simulink model "QD2_DroneStack_PID_2021a"  (R2022a)
settings: Solver=ode1  StartTime=0.0  StopTime=inf  FixedStep=1/1000  RelTol=1e-3  EnableMultiTasking=on
InitFcn:
  | Motor_Mapping_7_Inch
model workspace (MAT data in the model file):
  target_system = 1
values from neighbouring files (symbols this model uses):
  KT = [0.03616,0.117,-0.01215]    [Motor_Mapping_7_Inch.m]
  Motor_Matrix = [ 0.25   -1/(2*L_Roll)    1/(2*L_Pitch)    K_Tau/4;                  0.25   -1/(2*L_Roll)   -1/(2*L_Pitch)   -K_Tau/4;                  0.25    1/(2*L_Roll)    1/(2*L_Pitch)   -K_Tau/4;                  0.25    1/(2*L_Roll)   -1/(2*L_Pitch)    K_Tau/4]    [Motor_Mapping_7_Inch.m]
undefined symbols (not defined in the file or in its folder): _Commander, _QDrone2, _Stabilizer, datetime, HIL, lf, log_, m, n, qc_get_step_size, s, saved_data
libraries: quarc_library x94, simulink x27, simulink_extras x9
(part 3 of 4)

== system QD2_DroneStack_PID_2021a/COMMANDER (ANGLE MODE)/STATE MACHINE SIGNALS/Generate Extra Messages for Console ==
  time (s) : Inport
  Signal Triggers : Inport  Port=2
  Boolean Edge-Based Triggered Print : Subsystem  TreatAsAtomicUnit=on
  Matrix Concatenate : Concatenate  NumInputs=3  Mode=Multidimensional array  ConcatenateDimension=2
  String Constant12 : quarc_library/Strings/String Constant  string_value=DRONE DISARMED  evaluate_string=off  string_type=text  max_length=80  sample_time=inf  variable_size=off
      settings: AttributesFormatString="\"DRONE DISARMED\""  SourceProductName=QUARC Targets
  String Constant13 : quarc_library/Strings/String Constant  string_value=DRONE LANDING  evaluate_string=off  string_type=text  max_length=80  sample_time=inf  variable_size=off
      settings: AttributesFormatString="\"DRONE LANDING\""  SourceProductName=QUARC Targets
  String Constant16 : quarc_library/Strings/String Constant  string_value=INITIALIZATION FINISHED  evaluate_string=off  string_type=text  max_length=80  sample_time=inf  variable_size=off
      settings: AttributesFormatString="\"INITIALIZATION FINISHED\""  SourceProductName=QUARC Targets
  Terminator : Terminator
  wires:
  Boolean Edge-Based Triggered Print/1(Out1) -> Terminator/1
  String Constant13/1 -> Matrix Concatenate/3
  String Constant12/1 -> Matrix Concatenate/2
  String Constant16/1 -> Matrix Concatenate/1
  Signal Triggers/1 -> Boolean Edge-Based Triggered Print/1(Signal Enable)
  time (s)/1 -> Boolean Edge-Based Triggered Print/3(time (s))
  Matrix Concatenate/1 -> Boolean Edge-Based Triggered Print/2(Message)

== system QD2_DroneStack_PID_2021a/COMMANDER (ANGLE MODE)/STATE MACHINE SIGNALS/Generate State Messages for Console ==
  time (s) : Inport
  DroneState [1-9] : Inport  Port=2
  Detect Change : simulink/Logic and Bit Operations/Detect Change  vinit=0  OutDataTypeStr=boolean
  Multiport Switch : MultiPortSwitch  Inputs=9  SaturateOnIntegerOverflow=off  InputSameDT=off
  String Constant1 : quarc_library/Strings/String Constant  string_value=DRONE ARMED  evaluate_string=off  string_type=text  max_length=80  sample_time=inf  variable_size=off
      settings: AttributesFormatString="\"DRONE ARMED\""  SourceProductName=QUARC Targets
  String Constant2 : quarc_library/Strings/String Constant  string_value=DRONE TAKEOFF THROTTLE  evaluate_string=off  string_type=text  max_length=80  sample_time=inf  variable_size=off
      settings: AttributesFormatString="\"DRONE TAKEOFF THROTTLE\""  SourceProductName=QUARC Targets
  String Constant3 : quarc_library/Strings/String Constant  string_value=DRONE TAKEOFF HEIGHT STATE  evaluate_string=off  string_type=text  max_length=80  sample_time=inf  variable_size=off
      settings: AttributesFormatString="\"DRONE TAKEOFF HEIGHT STATE\""  SourceProductName=QUARC Targets
  String Constant4 : quarc_library/Strings/String Constant  string_value=ERROR - DRONE EMERGENCY STOP  evaluate_string=off  string_type=text  max_length=80  sample_time=inf  variable_size=off
      settings: AttributesFormatString="\"ERROR - DRONE EMERGENCY STOP\""  SourceProductName=QUARC Targets
  String Constant5 : quarc_library/Strings/String Constant  string_value=DRONE IDLE - WAITING TO BE ARMED  evaluate_string=off  string_type=text  max_length=80  sample_time=inf  variable_size=off
      settings: AttributesFormatString="\"DRONE IDLE - WAITING TO BE ARMED\""  SourceProductName=QUARC Targets
  String Constant6 : quarc_library/Strings/String Constant  string_value=DRONE IS IN FLIGHT STATE  evaluate_string=off  string_type=text  max_length=80  sample_time=inf  variable_size=off
      settings: AttributesFormatString="\"DRONE IS IN FLIGHT STATE\""  SourceProductName=QUARC Targets
  String Constant7 : quarc_library/Strings/String Constant  string_value=EMERGENCY STOP WAS PRESSED ON JOYSTICK  evaluate_string=off  string_type=text  max_length=80  sample_time=inf  variable_size=off
      settings: AttributesFormatString="\"EMERGENCY STOP WAS PRESSED ON JOYSTICK\""  SourceProductName=QUARC Targets
  String Constant8 : quarc_library/Strings/String Constant  string_value=FLIGHT FINISHED DRONE IS DISABLED  evaluate_string=off  string_type=text  max_length=80  sample_time=inf  variable_size=off
      settings: AttributesFormatString="\"FLIGHT FINISHED DRONE IS DISABLED\""  SourceProductName=QUARC Targets
  String Constant9 : quarc_library/Strings/String Constant  string_value=DRONE IS AUTO LANDING  evaluate_string=off  string_type=text  max_length=80  sample_time=inf  variable_size=off
      settings: AttributesFormatString="\"DRONE IS AUTO LANDING\""  SourceProductName=QUARC Targets
  Triggered Subsystem : Subsystem  TreatAsAtomicUnit=on
  wires:
  Detect Change/1 -> Triggered Subsystem/Trigger
  String Constant5/1 -> Multiport Switch/2
  String Constant8/1 -> Multiport Switch/10
  String Constant7/1 -> Multiport Switch/9
  String Constant4/1 -> Multiport Switch/8
  String Constant9/1 -> Multiport Switch/7
  String Constant6/1 -> Multiport Switch/6
  String Constant3/1 -> Multiport Switch/5
  String Constant2/1 -> Multiport Switch/4
  String Constant1/1 -> Multiport Switch/3
  time (s)/1 -> Triggered Subsystem/2(Time (s))
  Multiport Switch/1 -> Triggered Subsystem/3(Message)
  DroneState [1-9]/1 -> Detect Change/1, Triggered Subsystem/1(Value), Multiport Switch/1

== system QD2_DroneStack_PID_2021a/COMMANDER (ANGLE MODE)/STATE MACHINE SIGNALS/Generate Warning Messages for Console ==
  time (s) : Inport
  errors [8] : Inport  Port=2
  Boolean Value-Based Triggered Print : Subsystem  TreatAsAtomicUnit=on
  Matrix Concatenate : Concatenate  NumInputs=9  Mode=Multidimensional array  ConcatenateDimension=2
  String Constant : quarc_library/Strings/String Constant  string_value=Commander: Low Battery  evaluate_string=off  string_type=text  max_length=80  sample_time=inf  variable_size=off
      settings: AttributesFormatString="\"Commander: Low Battery\""  SourceProductName=QUARC Targets
  String Constant1 : quarc_library/Strings/String Constant  string_value=Commander: Sensor Failure  evaluate_string=off  string_type=text  max_length=80  sample_time=inf  variable_size=off
      settings: AttributesFormatString="\"Commander: Sensor Failure\""  SourceProductName=QUARC Targets
  String Constant2 : quarc_library/Strings/String Constant  string_value=Commander: Host Stream Issue / Problem with communication  evaluate_string=off  string_type=text  max_length=80  sample_time=inf  variable_size=off
      settings: AttributesFormatString="\"Commander: Host Stream Issue / Problem with communication\""  SourceProductName=QUARC Targets
  String Constant3 : quarc_library/Strings/String Constant  string_value=Commander: Joystick Issue  evaluate_string=off  string_type=text  max_length=80  sample_time=inf  variable_size=off
      settings: AttributesFormatString="\"Commander: Joystick Issue\""  SourceProductName=QUARC Targets
  String Constant4 : quarc_library/Strings/String Constant  string_value=Commander: Optitrack isn't tracking  evaluate_string=off  string_type=text  max_length=80  sample_time=inf  variable_size=off
      settings: AttributesFormatString="\"Commander: Optitrack isn't tracking\""  SourceProductName=QUARC Targets
  String Constant5 : quarc_library/Strings/String Constant  string_value=Commander: Flying low  evaluate_string=off  string_type=text  max_length=80  sample_time=inf  variable_size=off
      settings: AttributesFormatString="\"Commander: Flying low\""  SourceProductName=QUARC Targets
  String Constant6 : quarc_library/Strings/String Constant  string_value=Commander: Flying high  evaluate_string=off  string_type=text  max_length=80  sample_time=inf  variable_size=off
      settings: AttributesFormatString="\"Commander: Flying high\""  SourceProductName=QUARC Targets
  String Constant7 : quarc_library/Strings/String Constant  string_value=Commander: Emergency Stop Triggered  evaluate_string=off  string_type=text  max_length=80  sample_time=inf  variable_size=off
      settings: AttributesFormatString="\"Commander: Emergency Stop Triggered\""  SourceProductName=QUARC Targets
  String Constant8 : quarc_library/Strings/String Constant  string_value=Commander: Takeoff triggered before armed drone  evaluate_string=off  string_type=text  max_length=80  sample_time=inf  variable_size=off
      settings: AttributesFormatString="\"Commander: Takeoff triggered before armed drone\""  SourceProductName=QUARC Targets
  Terminator : Terminator
  wires:
  time (s)/1 -> Boolean Value-Based Triggered Print/3(time (s))
  errors [8]/1 -> Boolean Value-Based Triggered Print/1(Signal Enable)
  Matrix Concatenate/1 -> Boolean Value-Based Triggered Print/2(Message)
  String Constant/1 -> Matrix Concatenate/1
  String Constant1/1 -> Matrix Concatenate/2
  String Constant2/1 -> Matrix Concatenate/3
  String Constant3/1 -> Matrix Concatenate/4
  Boolean Value-Based Triggered Print/1(Out1) -> Terminator/1
  String Constant7/1 -> Matrix Concatenate/9
  String Constant6/1 -> Matrix Concatenate/8
  String Constant5/1 -> Matrix Concatenate/7
  String Constant4/1 -> Matrix Concatenate/6
  String Constant8/1 -> Matrix Concatenate/5

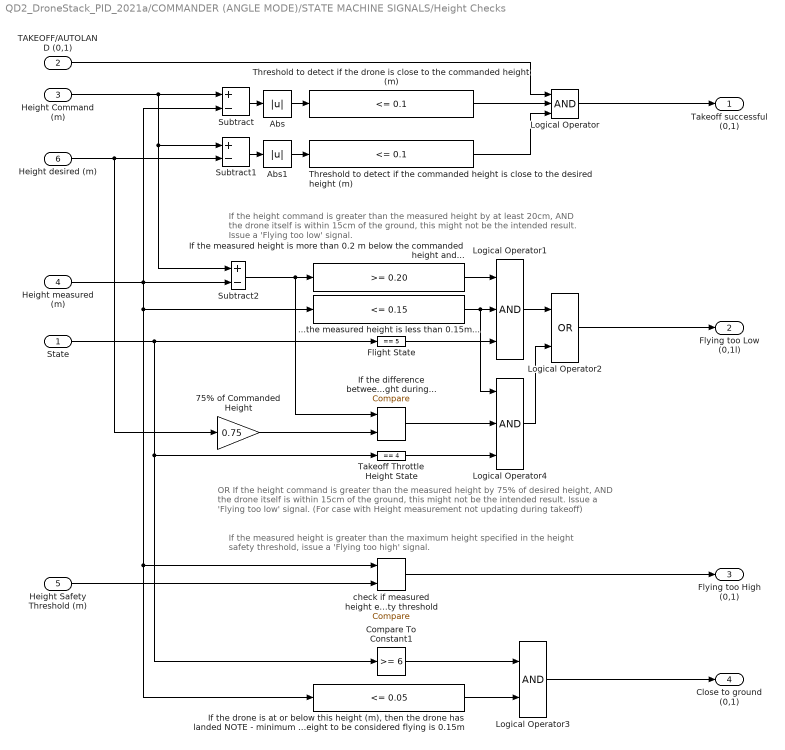
== system QD2_DroneStack_PID_2021a/COMMANDER (ANGLE MODE)/STATE MACHINE SIGNALS/Height Checks ==
  note: If the height command is greater than the measured height by at least 20cm, AND the drone itself is
      | within 15cm of the ground, this might not be the intended result. Issue a 'Flying too low' signal.
  note: If the measured height is greater than the maximum height specified in the height safety threshold,
      | issue a 'Flying too high' signal.
  note: OR If the height command is greater than the measured height by 75% of desired height, AND
      | the drone itself is within 15cm of the ground, this might not be the intended result. Issue a 'Flying too low' signal.
      | (For case with Height measurement not updating during takeoff)
  State : Inport
  TAKEOFF/AUTOLAND (0,1) : Inport  Port=2
  Height Command (m) : Inport  Port=3
  Height measured (m) : Inport  Port=4
  Height Safety Threshold (m) : Inport  Port=5
  Height desired (m) : Inport  Port=6
  ...the measured height is less than 0.15m... : simulink/Logic and Bit Operations/Compare To Constant  relop=<=  const=0.15  OutDataTypeStr=boolean
  75% of Commanded Height : Gain  Gain=0.75
  Abs : Abs  SaturateOnIntegerOverflow=off
  Abs1 : Abs  SaturateOnIntegerOverflow=off
  Compare To Constant1 : simulink/Logic and Bit Operations/Compare To Constant  relop=>=  const=6  OutDataTypeStr=boolean
  Flight State : simulink/Logic and Bit Operations/Compare To Constant  relop===  const=5  OutDataTypeStr=boolean
  If the difference between the measured and commanded height is greater than 75% of the commanded height during... : quarc_library/Logic Operations/Compare  operator=>=  output_data_type=boolean
      settings: SourceProductName=QUARC Targets
  "If the drone is at or below this height (m), then the drone has landed NOTE - minimum height to be considered flying is 0.15m   " : simulink/Logic and Bit Operations/Compare To Constant  relop=<=  const=0.05  OutDataTypeStr=boolean
  If the measured height is more than 0.2 m below the commanded height and... : simulink/Logic and Bit Operations/Compare To Constant  relop=>=  const=0.20  OutDataTypeStr=boolean
  Logical Operator : Logic  Inputs=3  AllPortsSameDT=off  OutDataTypeStr=boolean
  Logical Operator1 : Logic  Inputs=3  AllPortsSameDT=off  OutDataTypeStr=boolean
  Logical Operator2 : Logic  Operator=OR  AllPortsSameDT=off  OutDataTypeStr=boolean
  Logical Operator3 : Logic  AllPortsSameDT=off  OutDataTypeStr=boolean
  Logical Operator4 : Logic  Inputs=3  AllPortsSameDT=off  OutDataTypeStr=boolean
  Subtract : Sum  Inputs=+-
  Subtract1 : Sum  Inputs=+-
  Subtract2 : Sum  Inputs=+-
  Takeoff Throttle Height State : simulink/Logic and Bit Operations/Compare To Constant  relop===  const=4  OutDataTypeStr=boolean
  Threshold to detect if the commanded height is close to the desired height (m) : simulink/Logic and Bit Operations/Compare To Constant  relop=<=  const=0.1  OutDataTypeStr=boolean
  Threshold to detect if the drone is close to the commanded height (m) : simulink/Logic and Bit Operations/Compare To Constant  relop=<=  const=0.1  OutDataTypeStr=boolean
  check if measured height exceeds maximum height safety threshold : quarc_library/Logic Operations/Compare  operator=>=  output_data_type=boolean
      settings: SourceProductName=QUARC Targets
  Takeoff successful (0,1) : Outport  VectorParamsAs1DForOutWhenUnconnected=off
  Flying too Low (0,1l) : Outport  Port=2  VectorParamsAs1DForOutWhenUnconnected=off
  Flying too High (0,1) : Outport  Port=3  VectorParamsAs1DForOutWhenUnconnected=off
  Close to ground (0,1) : Outport  Port=4  VectorParamsAs1DForOutWhenUnconnected=off
  wires:
  Logical Operator/1 -> Takeoff successful (0,1)/1
  Logical Operator2/1 -> Flying too Low (0,1l)/1
  Subtract1/1 -> Abs1/1
  Threshold to detect if the commanded height is close to the desired height (m)/1 -> Logical Operator/3
  Abs/1 -> Threshold to detect if the drone is close to the commanded height (m)/1
  Threshold to detect if the drone is close to the commanded height (m)/1 -> Logical Operator/2
  Abs1/1 -> Threshold to detect if the commanded height is close to the desired height (m)/1
  Height desired (m)/1 -> 75% of Commanded Height/1, Subtract1/2
  TAKEOFF/AUTOLAND (0,1)/1 -> Logical Operator/1
  Subtract/1 -> Abs/1
  If the measured height is more than 0.2 m below the commanded height and.../1 -> Logical Operator1/1
  Logical Operator1/1 -> Logical Operator2/1
  Height Command (m)/1 -> Subtract1/1, Subtract2/1, Subtract/1
  ...the measured height is less than 0.15m.../1 -> Logical Operator4/1, Logical Operator1/2
  check if measured height exceeds maximum height safety threshold/1 -> Flying too High (0,1)/1
  Height Safety Threshold (m)/1 -> check if measured height exceeds maximum height safety threshold/2
  State/1 -> Flight State/1, Takeoff Throttle Height State/1, Compare To Constant1/1
  Logical Operator3/1 -> Close to ground (0,1)/1
  "If the drone is at or below this height (m), then the drone has landed NOTE - minimum height to be considered flying is 0.15m   "/1 -> Logical Operator3/2
  Compare To Constant1/1 -> Logical Operator3/1
  Height measured (m)/1 -> Subtract/2, ...the measured height is less than 0.15m.../1, "If the drone is at or below this height (m), then the drone has landed NOTE - minimum height to be considered flying is 0.15m   "/1, check if measured height exceeds maximum height safety threshold/1, Subtract2/2
  Logical Operator4/1 -> Logical Operator2/2
  Flight State/1 -> Logical Operator1/3
  Subtract2/1 -> If the difference between the measured and commanded height is greater than 75% of the commanded height during.../1, If the measured height is more than 0.2 m below the commanded height and.../1
  Takeoff Throttle Height State/1 -> Logical Operator4/3
  75% of Commanded Height/1 -> If the difference between the measured and commanded height is greater than 75% of the commanded height during.../2
  If the difference between the measured and commanded height is greater than 75% of the commanded height during.../1 -> Logical Operator4/2

== system QD2_DroneStack_PID_2021a/COMMANDER (ANGLE MODE)/STATE MACHINE SIGNALS/Latch E-Stop ==
  Input : Inport
  Trigger : TriggerPort  VariantControl=Variant
  Latched Output : Outport  InitialOutput=0  VectorParamsAs1DForOutWhenUnconnected=off
  wires:
  Input/1 -> Latched Output/1

== system QD2_DroneStack_PID_2021a/COMMANDER (ANGLE MODE)/STATE MACHINE SIGNALS/Throttle Checks ==
  Throttle Command (N) : Inport
  Controller Throttle Command (N) : Inport  Port=2
  Throttle Trim (N) : Inport  Port=3
  Max Thrust (N) : Inport  Port=4
  Abs : Abs  SaturateOnIntegerOverflow=off
  Abs1 : Abs  SaturateOnIntegerOverflow=off
  Compare : quarc_library/Logic Operations/Compare  operator=<=  output_data_type=boolean
      settings: SourceProductName=QUARC Targets
  Compare1 : quarc_library/Logic Operations/Compare  operator=<=  output_data_type=boolean
      settings: SourceProductName=QUARC Targets
  Compare2 : quarc_library/Logic Operations/Compare  operator=<=  output_data_type=boolean
      settings: SourceProductName=QUARC Targets
  "MAX throttle percentage (%) For CMD " : Constant  Value=0.171
  "MAX throttle percentage (%) For Ctrl " : Constant  Value=0.068
  "MAX throttle percentage (%) For Trim  " : Constant  Value=0.034
  Product : Product
  Product1 : Product
  Product2 : Product
  Subtract : Sum  Inputs=+-
  Threshold below which throttle can be assumed to be close to zero (N) (17.1% of Max Thrust) : simulink/Logic and Bit Operations/Compare To Constant  Commented=on  relop=<=  const=3.5  OutDataTypeStr=boolean
  Threshold to determine if the controller throttle is close to zero (N) (6.8% of Max Thrust) : simulink/Logic and Bit Operations/Compare To Constant  Commented=on  relop=<=  const=1.40  OutDataTypeStr=boolean
  Threshold to determine if throttle is close to the trim value (N) (3.4% of Max Thrust) : simulink/Logic and Bit Operations/Compare To Constant  Commented=on  relop=<=  const=0.7  OutDataTypeStr=boolean
  CMD Throttle at Trim (0,1) : Outport  VectorParamsAs1DForOutWhenUnconnected=off
  CMD Throttle close to 0 (0,1) : Outport  Port=2  VectorParamsAs1DForOutWhenUnconnected=off
  Ctrl Throttle close to 0 (0,1) : Outport  Port=3  VectorParamsAs1DForOutWhenUnconnected=off
  wires:
  Throttle Command (N)/1 -> Compare1/1, Subtract/1
  Throttle Trim (N)/1 -> Subtract/2
  Subtract/1 -> Abs/1
  Compare/1 -> CMD Throttle at Trim (0,1)/1
  Compare1/1 -> CMD Throttle close to 0 (0,1)/1
  Abs1/1 -> Compare2/1
  Controller Throttle Command (N)/1 -> Abs1/1
  Compare2/1 -> Ctrl Throttle close to 0 (0,1)/1
  "MAX throttle percentage (%) For Trim  "/1 -> Product1/1
  "MAX throttle percentage (%) For CMD "/1 -> Product/1
  "MAX throttle percentage (%) For Ctrl "/1 -> Product2/1
  Max Thrust (N)/1 -> Product1/2, Product/2, Product2/2
  Product1/1 -> Compare/2
  Abs/1 -> Compare/1
  Product/1 -> Compare1/2
  Product2/1 -> Compare2/2

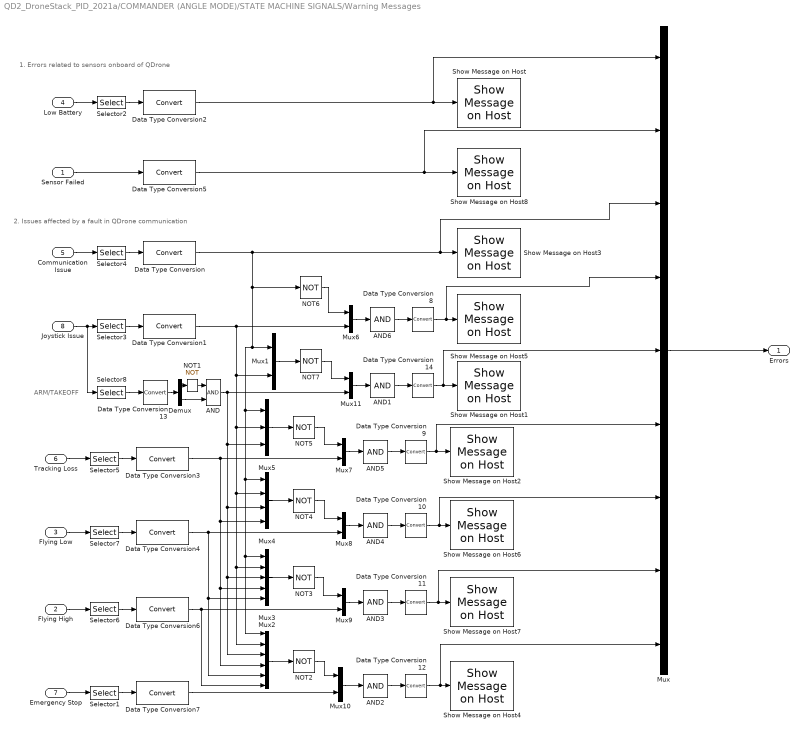
== system QD2_DroneStack_PID_2021a/COMMANDER (ANGLE MODE)/STATE MACHINE SIGNALS/Warning Messages ==
  note: ARM/TAKEOFF
  note: 1. Errors related to sensors onboard of QDrone
  note: 2. Issues affected by a fault in QDrone communication
  Sensor Failed : Inport
  Flying High : Inport  Port=2
  Flying Low : Inport  Port=3
  Low Battery : Inport  Port=4
  Communication Issue : Inport  Port=5
  Tracking Loss : Inport  Port=6
  "Emergency Stop " : Inport  Port=7
  Joystick Issue : Inport  Port=8
  AND : Logic  AllPortsSameDT=off  OutDataTypeStr=boolean
  AND{1..6} (6 alike) : Logic  Inputs=1  AllPortsSameDT=off  OutDataTypeStr=boolean
  Data Type Conversion{,1..14} (15 alike) : DataTypeConversion  SaturateOnIntegerOverflow=off  RndMeth=Floor
  Demux : Demux  Outputs=2
  Mux : Mux  Inputs=9
  Mux1 : Mux  Inputs=[1 1]
  Mux{6..11} (6 alike) : Mux  Inputs=2
  Mux2 : Mux  Inputs=[1 1 1 1 1 1]
  Mux3 : Mux  Inputs=[ 1 1 1 1 1]
  Mux4 : Mux  Inputs=[1 1 1 1]
  Mux5 : Mux  Inputs=[1 1 1]
  NOT{1..7} (7 alike) : Logic  Operator=NOT  IconShape=distinctive  AllPortsSameDT=off  OutDataTypeStr=boolean
  Selector1 : Selector  InputPortWidth=4  IndexOptions=Index vector (dialog)  Indices=3  OutputSizes=1
  Selector2 : Selector  InputPortWidth=5  IndexOptions=Index vector (dialog)  Indices=5  OutputSizes=1
  Selector3 : Selector  InputPortWidth=4  IndexOptions=Index vector (dialog)  Indices=4  OutputSizes=1
  Selector4 : Selector  InputPortWidth=5  IndexOptions=Index vector (dialog)  Indices=4  OutputSizes=1
  Selector5 : Selector  InputPortWidth=5  IndexOptions=Index vector (dialog)  Indices=3  OutputSizes=1
  Selector6 : Selector  InputPortWidth=4  IndexOptions=Index vector (dialog)  Indices=3  OutputSizes=1
  Selector7 : Selector  InputPortWidth=4  IndexOptions=Index vector (dialog)  Indices=2  OutputSizes=1
  Selector8 : Selector  InputPortWidth=4  IndexOptions=Index vector (dialog)  Indices=[1:2]  OutputSizes=1
  Show Message on Host : quarc_library/Sinks/Error Handling/Show Message on Host  message_type=Fixed error message  message_icon=Warning  message=Commander: Low Battery
      settings: AttributesFormatString="\"%<message>\""  SourceProductName=QUARC Targets
  Show Message on Host1 : quarc_library/Sinks/Error Handling/Show Message on Host  message_type=Fixed error message  message_icon=Warning  message=Commander: Takeoff triggered before armed drone
      settings: AttributesFormatString="\"%<message>\""  SourceProductName=QUARC Targets
  Show Message on Host2 : quarc_library/Sinks/Error Handling/Show Message on Host  message_type=Fixed error message  message_icon=Warning  message=Commander: Optitrack isn't tracking
      settings: AttributesFormatString="\"%<message>\""  SourceProductName=QUARC Targets
  Show Message on Host3 : quarc_library/Sinks/Error Handling/Show Message on Host  message_type=Fixed error message  message_icon=Warning  message=Commander: Host Stream Issue
      settings: AttributesFormatString="\"%<message>\""  SourceProductName=QUARC Targets
  Show Message on Host4 : quarc_library/Sinks/Error Handling/Show Message on Host  message_type=Fixed error message  message_icon=Warning  message=Commander: Emergency Stop Triggered
      settings: AttributesFormatString="\"%<message>\""  SourceProductName=QUARC Targets
  Show Message on Host5 : quarc_library/Sinks/Error Handling/Show Message on Host  message_type=Fixed error message  message_icon=Warning  message=Commander: Joystick Issue
      settings: AttributesFormatString="\"%<message>\""  SourceProductName=QUARC Targets
  Show Message on Host6 : quarc_library/Sinks/Error Handling/Show Message on Host  message_type=Fixed error message  message_icon=Warning  message=Commander: Flying low
      settings: AttributesFormatString="\"%<message>\""  SourceProductName=QUARC Targets
  Show Message on Host7 : quarc_library/Sinks/Error Handling/Show Message on Host  message_type=Fixed error message  message_icon=Warning  message=Commander: Flying high
      settings: AttributesFormatString="\"%<message>\""  SourceProductName=QUARC Targets
  Show Message on Host8 : quarc_library/Sinks/Error Handling/Show Message on Host  message_type=Fixed error message  message_icon=Warning  message=Commander: Sensor Failure
      settings: AttributesFormatString="\"%<message>\""  SourceProductName=QUARC Targets
  Errors : Outport
  wires:
  NOT2/1 -> Mux10/1
  Mux2/1 -> NOT2/1
  NOT3/1 -> Mux9/1
  Mux3/1 -> NOT3/1
  NOT4/1 -> Mux8/1
  Mux4/1 -> NOT4/1
  NOT5/1 -> Mux7/1
  Mux5/1 -> NOT5/1
  NOT6/1 -> Mux6/1
  Sensor Failed/1 -> Data Type Conversion5/1
  Selector6/1 -> Data Type Conversion6/1
  Selector1/1 -> Data Type Conversion7/1
  Low Battery/1 -> Selector2/1
  Communication Issue/1 -> Selector4/1
  "Emergency Stop "/1 -> Selector1/1
  AND2/1 -> Data Type Conversion12/1
  AND3/1 -> Data Type Conversion11/1
  AND4/1 -> Data Type Conversion10/1
  AND5/1 -> Data Type Conversion9/1
  AND6/1 -> Data Type Conversion8/1
  Selector2/1 -> Data Type Conversion2/1
  Selector3/1 -> Data Type Conversion1/1
  Selector4/1 -> Data Type Conversion/1
  Selector5/1 -> Data Type Conversion3/1
  Selector7/1 -> Data Type Conversion4/1
  Data Type Conversion3/1 -> Mux7/2, Mux4/4, Mux3/4, Mux2/4
  Data Type Conversion4/1 -> Mux8/2, Mux2/5, Mux3/5
  Data Type Conversion6/1 -> Mux2/6, Mux9/2
  Data Type Conversion7/1 -> Mux10/2
  Mux6/1 -> AND6/1
  Mux10/1 -> AND2/1
  Data Type Conversion12/1 -> Mux/9, Show Message on Host4/1
  Mux9/1 -> AND3/1
  Mux7/1 -> AND5/1
  Mux8/1 -> AND4/1
  Data Type Conversion2/1 -> Mux/1, Show Message on Host/1
  Data Type Conversion5/1 -> Mux/2, Show Message on Host8/1
  Tracking Loss/1 -> Selector5/1
  Flying Low/1 -> Selector7/1
  Flying High/1 -> Selector6/1
  Joystick Issue/1 -> Selector8/1, Selector3/1
  Data Type Conversion9/1 -> Mux/6, Show Message on Host2/1
  Data Type Conversion8/1 -> Mux/4, Show Message on Host5/1
  Data Type Conversion10/1 -> Mux/7, Show Message on Host6/1
  Data Type Conversion11/1 -> Mux/8, Show Message on Host7/1
  Mux/1 -> Errors/1
  Selector8/1 -> Data Type Conversion13/1
  Data Type Conversion13/1 -> Demux/1
  Demux/1 -> NOT1/1
  Demux/2 -> AND/2
  NOT1/1 -> AND/1
  NOT7/1 -> Mux11/1
  Data Type Conversion14/1 -> Mux/5, Show Message on Host1/1
  AND1/1 -> Data Type Conversion14/1
  Data Type Conversion1/1 -> Mux6/2, Mux1/2, Mux5/2, Mux4/2, Mux3/2, Mux2/2
  Mux11/1 -> AND1/1
  Data Type Conversion/1 -> NOT6/1, Mux1/1, Mux5/1, Mux4/1, Mux3/1, Mux2/1, Mux/3, Show Message on Host3/1
  Mux1/1 -> NOT7/1
  AND/1 -> Mux2/3, Mux3/3, Mux4/3, Mux5/3, Mux11/2

== system QD2_DroneStack_PID_2021a/COMMANDER (ANGLE MODE)/THROTTLE SWITCHBOX /Use desired height when enabled ==
  h_d (m) [1] : Inport
  Enable : EnablePort
  Out1 : Outport  OutputWhenDisabled=reset  InitialOutput=0  VectorParamsAs1DForOutWhenUnconnected=off
  wires:
  h_d (m) [1]/1 -> Out1/1

== system QD2_DroneStack_PID_2021a/HORIZON FRAME CONVERSION AND ESTIMATION/Pose Switchbox/Use des height when enabled ==
  h_d (m) [1] : Inport
  Enable : EnablePort
  Out1 : Outport  OutputWhenDisabled=reset  InitialOutput=0  VectorParamsAs1DForOutWhenUnconnected=off
  wires:
  h_d (m) [1]/1 -> Out1/1

== system QD2_DroneStack_PID_2021a/HORIZON FRAME CONVERSION AND ESTIMATION/Pose Switchbox/Use des yaw when enabled ==
  h_d (m) [1] : Inport
  Enable : EnablePort
  Out1 : Outport  OutputWhenDisabled=reset  InitialOutput=0  VectorParamsAs1DForOutWhenUnconnected=off
  wires:
  h_d (m) [1]/1 -> Out1/1

== system QD2_DroneStack_PID_2021a/HORIZON FRAME CONVERSION AND ESTIMATION/Pose Switchbox/Use desired X when enabled ==
  h_d (m) [1] : Inport
  Enable : EnablePort
  Out1 : Outport  OutputWhenDisabled=reset  InitialOutput=0  VectorParamsAs1DForOutWhenUnconnected=off
  wires:
  h_d (m) [1]/1 -> Out1/1

== system QD2_DroneStack_PID_2021a/HORIZON FRAME CONVERSION AND ESTIMATION/Pose Switchbox/Use desired Y when enabled ==
  h_d (m) [1] : Inport
  Enable : EnablePort
  Out1 : Outport  OutputWhenDisabled=reset  InitialOutput=0  VectorParamsAs1DForOutWhenUnconnected=off
  wires:
  h_d (m) [1]/1 -> Out1/1

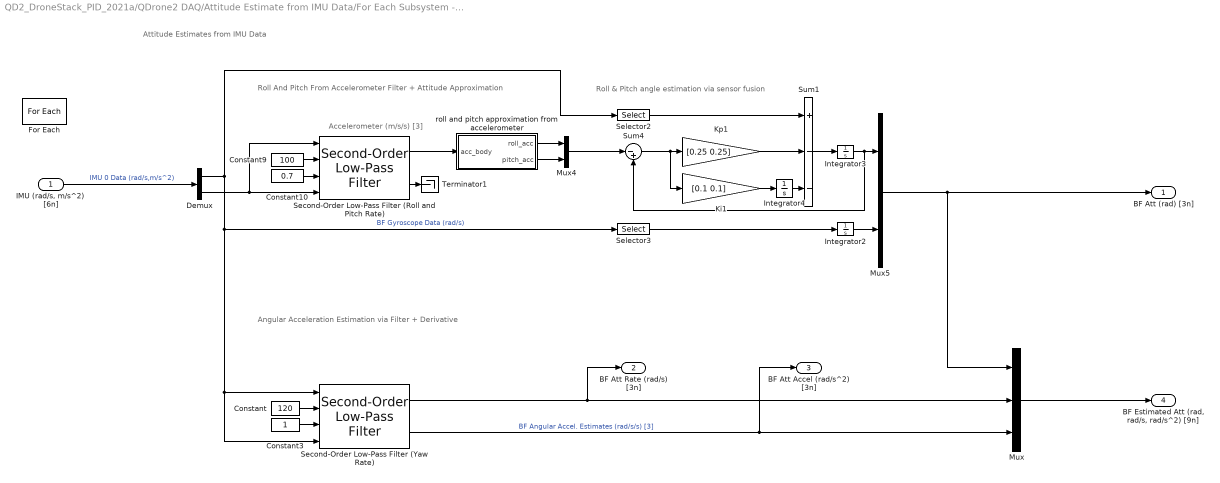
== system QD2_DroneStack_PID_2021a/QDrone2 DAQ/Attitude Estimate from IMU Data/For Each Subsystem - Attitutde Estimates ==
  note: Attitude Estimates from IMU Data
  note: Accelerometer (m/s/s) [3]
  note: Roll And Pitch From Accelerometer Filter + Attitude Approximation
  note: Roll & Pitch angle estimation via sensor fusion
  note: Angular Acceleration Estimation via Filter + Derivative
  "IMU (rad/s, m/s^2) [6n]" : Inport  Partition=on  PartitionDimension=1  PartitionWidth=6  PartitionOffset=0
  Constant : Constant  Value=120
  Constant10 : Constant  Value=0.7
  Constant3 : Constant
  Constant9 : Constant  Value=100
  Demux : Demux  Outputs=[3,3]
  For Each : ForEach  DisableCoverage=on
  Integrator2 : Integrator
  Integrator3 : Integrator
  Integrator4 : Integrator
  Ki1 : Gain  Gain=[0.1 0.1]
  Kp1 : Gain  Gain=[0.25 0.25]
  Mux : Mux  Inputs=3
  Mux4 : Mux  Inputs=2
  Mux5 : Mux  Inputs=2
  Second-Order Low-Pass Filter (Roll and Pitch Rate) : quarc_library/Continuous/Second-Order Low-Pass Filter  params_source=External (input ports)  input_width=200  input_zeta=1  input_init=0
  Second-Order Low-Pass Filter (Yaw Rate) : quarc_library/Continuous/Second-Order Low-Pass Filter  params_source=External (input ports)  input_width=200  input_zeta=1  input_init=0
  Selector2 : Selector  InputPortWidth=3  IndexOptions=Index vector (dialog)  Indices=[1,2]  OutputSizes=1
  Selector3 : Selector  InputPortWidth=3  IndexOptions=Index vector (dialog)  Indices=[3]  OutputSizes=1
  Sum1 : Sum  Inputs=+--
  Sum4 : Sum  Inputs=|-+
  Terminator1 : Terminator
  roll and pitch approximation from accelerometer : MATLAB Function  TreatAsAtomicUnit=on
  BF Att (rad) [3n] : Outport  ConcatenationDimension=1
  BF Att Rate (rad/s) [3n] : Outport  Port=2  ConcatenationDimension=1
  BF Att Accel (rad/s^2) [3n] : Outport  Port=3  ConcatenationDimension=1
  "BF Estimated Att (rad, rad/s, rad/s^2) [9n] " : Outport  Port=4  ConcatenationDimension=1
  wires:
  roll and pitch approximation from accelerometer/2(pitch_acc) -> Mux4/2
  Constant9/1 -> Second-Order Low-Pass Filter (Roll and Pitch Rate)/2
  Second-Order Low-Pass Filter (Roll and Pitch Rate)/1 -> roll and pitch approximation from accelerometer/1(acc_body)
  "IMU (rad/s, m/s^2) [6n]"/1 -> Demux/1  "IMU 0 Data (rad/s,m/s^2)"
  Constant10/1 -> Second-Order Low-Pass Filter (Roll and Pitch Rate)/3
  Demux/2 -> Second-Order Low-Pass Filter (Roll and Pitch Rate)/4, Second-Order Low-Pass Filter (Roll and Pitch Rate)/1
  Second-Order Low-Pass Filter (Roll and Pitch Rate)/2 -> Terminator1/1
  Selector3/1 -> Integrator2/1
  Integrator2/1 -> Mux5/2
  Integrator4/1 -> Sum1/3
  Kp1/1 -> Sum1/2
  Selector2/1 -> Sum1/1
  Integrator3/1 -> Sum4/2, Mux5/1
  Mux5/1 -> BF Att (rad) [3n]/1, Mux/1
  Sum4/1 -> Ki1/1, Kp1/1
  Sum1/1 -> Integrator3/1
  Ki1/1 -> Integrator4/1
  roll and pitch approximation from accelerometer/1(roll_acc) -> Mux4/1
  Mux4/1 -> Sum4/1
  Constant3/1 -> Second-Order Low-Pass Filter (Yaw Rate)/3
  Demux/1 -> Second-Order Low-Pass Filter (Yaw Rate)/4, Second-Order Low-Pass Filter (Yaw Rate)/1, Selector3/1, Selector2/1  "BF Gyroscope Data (rad/s)"
  Constant/1 -> Second-Order Low-Pass Filter (Yaw Rate)/2
  Second-Order Low-Pass Filter (Yaw Rate)/1 -> Mux/2, BF Att Rate (rad/s) [3n]/1
  Second-Order Low-Pass Filter (Yaw Rate)/2 -> BF Att Accel (rad/s^2) [3n]/1, Mux/3  "BF Angular Accel. Estimates (rad/s/s) [3]"
  Mux/1 -> "BF Estimated Att (rad, rad/s, rad/s^2) [9n] "/1

== system QD2_DroneStack_PID_2021a/QDrone2 DAQ/Check Battery level/Triggered Subsystem ==
  Trigger : TriggerPort  VariantControl=(inherit)
  Constant : Constant
  Out1 : Outport  InitialOutput=[0]
  wires:
  Constant/1 -> Out1/1

== system QD2_DroneStack_PID_2021a/QDrone2 DAQ/Sensor Failure Monitoring - IMU0/Sensor Failure (Accelerometer) ==
  note: Check for flat-line ZERO Accelerometer data (no data)
  Sensor Input : Inport
  Clock : Clock
  Compare To Constant : simulink/Logic and Bit Operations/Compare To Constant  relop=>=  const=1  OutDataTypeStr=boolean
  Demux1 : Demux  Outputs=3
  Logical Operator : Logic  Operator=OR  Inputs=3  AllPortsSameDT=off  OutDataTypeStr=boolean
  Logical Operator1 : Logic  AllPortsSameDT=off  OutDataTypeStr=boolean
  Terminator1 : Terminator
  Terminator3 : Terminator
  Terminator4 : Terminator
  Threshold : quarc_library/Discontinuities/Threshold  operator===  param_src=Specify via dialog  threshold=0  duration=1
      settings: SourceProductName=QUARC Targets
  Threshold1 : quarc_library/Discontinuities/Threshold  operator===  param_src=Specify via dialog  threshold=0  duration=1
      settings: SourceProductName=QUARC Targets
  Threshold2 : quarc_library/Discontinuities/Threshold  operator===  param_src=Specify via dialog  threshold=0  duration=1
      settings: SourceProductName=QUARC Targets
  Sensor Fault : Outport  VectorParamsAs1DForOutWhenUnconnected=off
  wires:
  Clock/1 -> Compare To Constant/1
  Threshold/1 -> Logical Operator/1
  Threshold1/1 -> Logical Operator/2
  Compare To Constant/1 -> Logical Operator1/1
  Logical Operator1/1 -> Sensor Fault/1
  Sensor Input/1 -> Demux1/1
  Threshold2/2 -> Terminator4/1
  Threshold2/1 -> Logical Operator/3
  Demux1/1 -> Threshold/1
  Demux1/3 -> Threshold2/1
  Demux1/2 -> Threshold1/1
  Logical Operator/1 -> Logical Operator1/2
  Threshold1/2 -> Terminator3/1
  Threshold/2 -> Terminator1/1

== system QD2_DroneStack_PID_2021a/QDrone2 DAQ/Sensor Failure Monitoring - IMU0/Sensor Failure (Gyroscope) ==
  note: Check for flat-line ZERO Gyro data (no data)
  Sensor Input : Inport
  Clock : Clock
  Compare To Constant : simulink/Logic and Bit Operations/Compare To Constant  relop=>=  const=1  OutDataTypeStr=boolean
  Demux1 : Demux  Outputs=3
  Logical Operator : Logic  Operator=OR  Inputs=3  AllPortsSameDT=off  OutDataTypeStr=boolean
  Logical Operator1 : Logic  AllPortsSameDT=off  OutDataTypeStr=boolean
  Terminator1 : Terminator
  Terminator3 : Terminator
  Terminator4 : Terminator
  Threshold : quarc_library/Discontinuities/Threshold  operator===  param_src=Specify via dialog  threshold=0  duration=1
      settings: SourceProductName=QUARC Targets
  Threshold1 : quarc_library/Discontinuities/Threshold  operator===  param_src=Specify via dialog  threshold=0  duration=1
      settings: SourceProductName=QUARC Targets
  Threshold2 : quarc_library/Discontinuities/Threshold  operator===  param_src=Specify via dialog  threshold=0  duration=1
      settings: SourceProductName=QUARC Targets
  Sensor Fault : Outport  VectorParamsAs1DForOutWhenUnconnected=off
  wires:
  Threshold/2 -> Terminator1/1
  Threshold1/2 -> Terminator3/1
  Logical Operator/1 -> Logical Operator1/2
  Demux1/2 -> Threshold1/1
  Demux1/3 -> Threshold2/1
  Demux1/1 -> Threshold/1
  Threshold2/1 -> Logical Operator/3
  Threshold2/2 -> Terminator4/1
  Sensor Input/1 -> Demux1/1
  Logical Operator1/1 -> Sensor Fault/1
  Compare To Constant/1 -> Logical Operator1/1
  Threshold1/1 -> Logical Operator/2
  Threshold/1 -> Logical Operator/1
  Clock/1 -> Compare To Constant/1

== system QD2_DroneStack_PID_2021a/QDrone2 DAQ/Sensor Failure Monitoring - IMU1/Sensor Failure (Accelerometer) ==
  note: Check for flat-line ZERO Accelerometer data (no data)
  Sensor Input : Inport
  Clock : Clock
  Compare To Constant : simulink/Logic and Bit Operations/Compare To Constant  relop=>=  const=1  OutDataTypeStr=boolean
  Demux1 : Demux  Outputs=3
  Logical Operator : Logic  Operator=OR  Inputs=3  AllPortsSameDT=off  OutDataTypeStr=boolean
  Logical Operator1 : Logic  AllPortsSameDT=off  OutDataTypeStr=boolean
  Terminator1 : Terminator
  Terminator3 : Terminator
  Terminator4 : Terminator
  Threshold : quarc_library/Discontinuities/Threshold  operator===  param_src=Specify via dialog  threshold=0  duration=1
      settings: SourceProductName=QUARC Targets
  Threshold1 : quarc_library/Discontinuities/Threshold  operator===  param_src=Specify via dialog  threshold=0  duration=1
      settings: SourceProductName=QUARC Targets
  Threshold2 : quarc_library/Discontinuities/Threshold  operator===  param_src=Specify via dialog  threshold=0  duration=1
      settings: SourceProductName=QUARC Targets
  Sensor Fault : Outport  VectorParamsAs1DForOutWhenUnconnected=off
  wires:
  Threshold/2 -> Terminator1/1
  Threshold1/2 -> Terminator3/1
  Logical Operator/1 -> Logical Operator1/2
  Demux1/2 -> Threshold1/1
  Demux1/3 -> Threshold2/1
  Demux1/1 -> Threshold/1
  Threshold2/1 -> Logical Operator/3
  Threshold2/2 -> Terminator4/1
  Sensor Input/1 -> Demux1/1
  Logical Operator1/1 -> Sensor Fault/1
  Compare To Constant/1 -> Logical Operator1/1
  Threshold1/1 -> Logical Operator/2
  Threshold/1 -> Logical Operator/1
  Clock/1 -> Compare To Constant/1

== system QD2_DroneStack_PID_2021a/QDrone2 DAQ/Sensor Failure Monitoring - IMU1/Sensor Failure (Gyroscope) ==
  note: Check for flat-line ZERO Gyro data (no data)
  Sensor Input : Inport
  Clock : Clock
  Compare To Constant : simulink/Logic and Bit Operations/Compare To Constant  relop=>=  const=1  OutDataTypeStr=boolean
  Demux1 : Demux  Outputs=3
  Logical Operator : Logic  Operator=OR  Inputs=3  AllPortsSameDT=off  OutDataTypeStr=boolean
  Logical Operator1 : Logic  AllPortsSameDT=off  OutDataTypeStr=boolean
  Terminator1 : Terminator
  Terminator3 : Terminator
  Terminator4 : Terminator
  Threshold : quarc_library/Discontinuities/Threshold  operator===  param_src=Specify via dialog  threshold=0  duration=1
      settings: SourceProductName=QUARC Targets
  Threshold1 : quarc_library/Discontinuities/Threshold  operator===  param_src=Specify via dialog  threshold=0  duration=1
      settings: SourceProductName=QUARC Targets
  Threshold2 : quarc_library/Discontinuities/Threshold  operator===  param_src=Specify via dialog  threshold=0  duration=1
      settings: SourceProductName=QUARC Targets
  Sensor Fault : Outport  VectorParamsAs1DForOutWhenUnconnected=off
  wires:
  Clock/1 -> Compare To Constant/1
  Threshold/1 -> Logical Operator/1
  Threshold1/1 -> Logical Operator/2
  Compare To Constant/1 -> Logical Operator1/1
  Logical Operator1/1 -> Sensor Fault/1
  Sensor Input/1 -> Demux1/1
  Threshold2/2 -> Terminator4/1
  Threshold2/1 -> Logical Operator/3
  Demux1/1 -> Threshold/1
  Demux1/3 -> Threshold2/1
  Demux1/2 -> Threshold1/1
  Logical Operator/1 -> Logical Operator1/2
  Threshold1/2 -> Terminator3/1
  Threshold/2 -> Terminator1/1

== system QD2_DroneStack_PID_2021a/QDrone2 DAQ/Subsystem1/Maintain previous value4 ==
  Value in : Inport
  Memory : Memory
  Switch : Switch  Criteria=u2 ~= 0  SaturateOnIntegerOverflow=off  InputSameDT=off
  Non 0 values : Outport
  wires:
  Value in/1 -> Switch/1, Switch/2
  Switch/1 -> Memory/1, Non 0 values/1
  Memory/1 -> Switch/3

== system QD2_DroneStack_PID_2021a/COMMANDER (ANGLE MODE)/STATE MACHINE SIGNALS/Generate Extra Messages for Console/Boolean Edge-Based Triggered Print ==
  Signal Enable : Inport  Partition=on  PartitionDimension=1  PartitionWidth=1  PartitionOffset=0
  Message : Inport  Port=2  Partition=on  PartitionDimension=2  PartitionWidth=1  PartitionOffset=0
  time (s) : Inport  Port=3
  For Each : ForEach  DisableCoverage=on
  Triggered Subsystem1 : Subsystem  TreatAsAtomicUnit=on
  Out1 : Outport  ConcatenationDimension=1
  wires:
  time (s)/1 -> Triggered Subsystem1/1(Time (s))
  Message/1 -> Triggered Subsystem1/2(Message)
  Signal Enable/1 -> Out1/1, Triggered Subsystem1/Trigger

== system QD2_DroneStack_PID_2021a/COMMANDER (ANGLE MODE)/STATE MACHINE SIGNALS/Generate State Messages for Console/Triggered Subsystem ==
  Value : Inport
  Time (s) : Inport  Port=2
  Message : Inport  Port=3
  Trigger : TriggerPort  VariantControl=(inherit)
  Data Type Conversion : DataTypeConversion  OutDataTypeStr=uint8  SaturateOnIntegerOverflow=off  RndMeth=Floor
  Print : quarc_library/User Interface/Standard I//O/Print  format_string="[ %lf ] (s): State %u  => %s \\n"  max_code_units=512  optimization=Minimizing latency  sample_time=-1  active=off
      settings: SourceProductName=QUARC Targets
  Terminator : Terminator
  Terminator1 : Terminator
  wires:
  Time (s)/1 -> Print/1
  Message/1 -> Print/3
  Print/2 -> Terminator/1
  Print/1 -> Terminator1/1
  Value/1 -> Data Type Conversion/1
  Data Type Conversion/1 -> Print/2

== system QD2_DroneStack_PID_2021a/COMMANDER (ANGLE MODE)/STATE MACHINE SIGNALS/Generate Warning Messages for Console/Boolean Value-Based Triggered Print ==
  Signal Enable : Inport  Partition=on  PartitionDimension=1  PartitionWidth=1  PartitionOffset=0
  Message : Inport  Port=2  Partition=on  PartitionDimension=2  PartitionWidth=1  PartitionOffset=0
  time (s) : Inport  Port=3
  For Each : ForEach  DisableCoverage=on
  Triggered Subsystem : Subsystem  TreatAsAtomicUnit=on
  Out1 : Outport  ConcatenationDimension=1
  wires:
  time (s)/1 -> Triggered Subsystem/1(Time (s))
  Message/1 -> Triggered Subsystem/2(Message)
  Signal Enable/1 -> Triggered Subsystem/Trigger, Out1/1

== system QD2_DroneStack_PID_2021a/COMMANDER (ANGLE MODE)/STATE MACHINE SIGNALS/Generate Extra Messages for Console/Boolean Edge-Based Triggered Print/Triggered Subsystem1 ==
  Time (s) : Inport
  Message : Inport  Port=2
  Trigger : TriggerPort  TriggerType=falling  VariantControl=(inherit)
  Print : quarc_library/User Interface/Standard I//O/Print  format_string=[ %lf ] (s): %s !\n  max_code_units=512  optimization=Minimizing latency  sample_time=-1  active=off
      settings: SourceProductName=QUARC Targets
  Terminator : Terminator
  Terminator1 : Terminator
  wires:
  Time (s)/1 -> Print/1
  Message/1 -> Print/2
  Print/2 -> Terminator/1
  Print/1 -> Terminator1/1

== system QD2_DroneStack_PID_2021a/COMMANDER (ANGLE MODE)/STATE MACHINE SIGNALS/Generate Warning Messages for Console/Boolean Value-Based Triggered Print/Triggered Subsystem ==
  Time (s) : Inport
  Message : Inport  Port=2
  Trigger : TriggerPort  VariantControl=(inherit)
  Print : quarc_library/User Interface/Standard I//O/Print  format_string=[ %lf ] (s): %s\n  max_code_units=512  optimization=Minimizing latency  sample_time=-1  active=off
      settings: SourceProductName=QUARC Targets
  Terminator : Terminator
  Terminator1 : Terminator
  wires:
  Print/1 -> Terminator1/1
  Print/2 -> Terminator/1
  Message/1 -> Print/2
  Time (s)/1 -> Print/1

== matlab function QD2_DroneStack_PID_2021a/HORIZON FRAME CONVERSION AND ESTIMATION/Pose Switchbox/MATLAB Function2 ==
  data: sigmoid_type input; enable output; height_des input; slow_lim input; fast_lim input; height_cur input; height_vel input; height_ref output; max_height_vel output; max_height_accel output
function [enable, height_ref, max_height_vel, max_height_accel] = fcn(sigmoid_type, height_des, slow_lim, fast_lim, height_cur, height_vel)

% Note: Some of the cases below are identical. However, they are separated out 
% based on the states of the state machine for ease of modification in the future. 
% For example, states 4 and 5 are identical. However, if the user wants different 
% signmoid behaviour when taking off than when landing, these cases may not be the same. 

enable = 0;
height_ref = 0;
max_height_vel = 0;
max_height_accel = 0;

switch sigmoid_type
    case 1 % This is for the IDLE, ARM, E_ABORT, E_STOP and DISABLE states of the FSM
        enable = 0;
        height_ref = 0;
        max_height_vel = 0;
        max_height_accel = 0;

    case 2 % This is for the TAKEOFF THROTTLE state of the FSM
        enable = 0;
        height_ref = 0;
        max_height_vel = 0;
        max_height_accel = 0;

    case 3 % This is for the FLIGHT state of the FSM 
        enable = 1;
        height_ref = height_des;
        max_height_vel = fast_lim(1);
        max_height_accel = fast_lim(2);

    case 4 % This is for the TAKEOFF HEIGHT state of the FSM
        enable = 1;
        height_ref = height_des;
        if (height_vel < 0)||(abs(height_cur - height_des) <= 0.1)||(height_des <= height_cur)
            max_height_vel = fast_lim(1);
            max_height_accel = fast_lim(2);
        else    
            max_height_vel = slow_lim(1);
            max_height_accel = slow_lim(2);
        end
    case 5 % This is for the AUTOLAND state of the FSM
        enable = 1;
        height_ref = 0;
        if height_vel >= 0
            max_height_vel = fast_lim(1);
            max_height_accel = fast_lim(2);        
        else
            max_height_vel = slow_lim(1);
            max_height_accel = slow_lim(2);
        end
        
end

== matlab function QD2_DroneStack_PID_2021a/HORIZON FRAME CONVERSION AND ESTIMATION/Pose Switchbox/MATLAB Function4 ==
  data: sigmoid_type input; enable output; yaw_des input; slow_lim input; fast_lim input; yaw_cur input; yaw_ref output; max_yaw_vel output; max_yaw_accel output; yaw_vel input
function [enable, yaw_ref, max_yaw_vel, max_yaw_accel] = fcn(sigmoid_type, yaw_des, slow_lim, fast_lim, yaw_cur, yaw_vel)

% Note: Some of the cases below are identical. However, they are separated out 
% based on the states of the state machine for ease of modification in the future. 
% For example, states 4 and 5 are identical. However, if the user wants different 
% signmoid behaviour when taking off than when landing, these cases may not be the same. 

enable = 0;
yaw_ref = 0;
max_yaw_vel = 0;
max_yaw_accel = 0;

switch sigmoid_type
    case 1 % This is for the IDLE, ARM, E_ABORT, E_STOP and DISABLE states of the FSM
        enable = 0;
        yaw_ref = 0;
        max_yaw_vel = 0;
        max_yaw_accel = 0;
    case 2 % This is for the TAKEOFF THROTTLE state of the FSM
        enable = 1;
        yaw_ref = yaw_des;
        max_yaw_vel = slow_lim(1);
        max_yaw_accel = slow_lim(2);  
    case 3 % This is for the FLIGHT state of the FSM 
        enable = 1;
        yaw_ref = yaw_des;
        max_yaw_vel = fast_lim(1);
        max_yaw_accel = fast_lim(2);
    case 4 % This is for the TAKEOFF HEIGHT state of the FSM
        enable = 1;
        yaw_ref = yaw_des;
        if (yaw_vel < 0)||(yaw_des < yaw_cur)||(abs(yaw_cur-yaw_des)<=0.2)
            max_yaw_vel = fast_lim(1);
            max_yaw_accel = fast_lim(2);
        else    
            max_yaw_vel = slow_lim(1);
            max_yaw_accel = slow_lim(2);
        end
    case 5 % This is for the AUTOLAND state of the FSM
        enable = 1;
        yaw_ref = yaw_des;
        if (yaw_vel >= 0)
            max_yaw_vel = fast_lim(1);
            max_yaw_accel = fast_lim(2);
        else    
            max_yaw_vel = slow_lim(1);
            max_yaw_accel = slow_lim(2);
        end
end

== matlab function QD2_DroneStack_PID_2021a/HORIZON FRAME CONVERSION AND ESTIMATION/Pose Switchbox/Signmoid Type ==
  data: FSM_state input; sigmoid_type output
function sigmoid_type  = sigmoid_type_position(FSM_state)

% QDrone: Position Switchbox
%
% Switching between different sigmoid types based on 
% which state the FSM is in.
%
% v3.0 - 4th October, 2018
%
% INPUTS:
% -------
% FSM_state = current state of the FSM------------------------------------------------------- (#)         [1]
% 
% OUTPUTS:
% --------
% sigmoid_type = an integer whose state determines how the commands/measurements are transformed-- (#)         [1]

% Sigmoid_type = 1; This is for the IDLE, ARM, E_ABORT, E_STOP and DISABLE states of the FSM
% Sigmoid_type = 2; This is for the TAKEOFF THROTTLE state of the FSM
% Sigmoid_type = 3; This is for the FLIGHT state of the FSM
% Sigmoid_type = 4; This is for the TAKEOFF HEIGHT state of the FSM
% Sigmoid_type = 5; This is for the AUTOLAND state of the FSM

sigmoid_type = 0;

switch FSM_state
    case 1 % IDLE STATE
        sigmoid_type = 1;
    case 2 % ARM STATE
        sigmoid_type = 1;
    case 3 % TAKEOFF THROTTLE STATE
        sigmoid_type = 2;
    case 4 % TAKEOFF HEIGHT STATE
        sigmoid_type = 4;
    case 5 % FLIGHT STATE
        sigmoid_type = 3;
    case 6 % AUTOLAND STATE
        sigmoid_type = 5;
    case 7 % EMERGENCY STOP STATE
        sigmoid_type = 1;
    case 8 % EMERGENCY ABORT STATE
        sigmoid_type = 1;
    case 9 % DISABLE STATE
        sigmoid_type = 1;
end

== matlab function QD2_DroneStack_PID_2021a/COMMANDER (ANGLE MODE)/THROTTLE SWITCHBOX /Hover Throttle Sigmoid Parameters ==
  data: sigmoid_type input; enable output; trim_throttle input; takeoff_lim input; land_lim input; throttle_vel input; throttle_ref output; max_throttle_vel output; max_throttle_accel output
function [enable, throttle_ref, max_throttle_vel, max_throttle_accel] = fcn(sigmoid_type, trim_throttle, takeoff_lim, land_lim, throttle_vel)

% Note: Some of the cases below are identical. However, they are separated out 
% based on the states of the state machine for ease of modification in the future. 
% For example, states 4 and 5 are identical. However, if the user wants different 
% signmoid behaviour when taking off than when landing, these cases may not be the same. 

enable = 0;
throttle_ref = 0;
max_throttle_vel = 0;
max_throttle_accel = 0;

switch sigmoid_type
    case 1 % sigmoid = 1 - Command 0 throttle
        % This is for the IDLE, ARM, E_ABORT, and DISABLE states of the FSM
        enable = 0;
        throttle_ref = 0;
        max_throttle_vel = 0;
        max_throttle_accel = 0;

    case 2 % sigmoid = 2 - Sigmoid throttle up from 0 to the trim value
        % This is for the TAKEOFF THROTTLE state of the FSM
        enable = 1;
        throttle_ref = trim_throttle;
        max_throttle_vel = takeoff_lim(1);
        max_throttle_accel = takeoff_lim(2);

    case 3 % sigmoid = 3 - Pass controller throttle straight through + trim value.
        % This is for the TAKEOFF HEIGHT and FLIGHT state of the FSM
        enable = 1;
        throttle_ref = trim_throttle;
        max_throttle_vel = takeoff_lim(1);
        max_throttle_accel = takeoff_lim(2);

    case 4 % sigmoid = 4 - Ignore controller throttle. Sigmoid it down to 0.
        % This is for the E_Landing state of the FSM
        enable = 1;
        throttle_ref = 0;
        if throttle_vel > 0
            max_throttle_vel = takeoff_lim(1);
            max_throttle_accel = takeoff_lim(2);
        else
            max_throttle_vel = land_lim(1);
            max_throttle_accel = land_lim(2);
        end
        
    case 5 % sigmoid = 5 - Pass controller throttle straight through + trim value.
        % This is for the AUTOLAND state of the FSM
        enable = 1;
        throttle_ref = trim_throttle;
        max_throttle_vel = takeoff_lim(1);
        max_throttle_accel = takeoff_lim(2);

end
